simulink model "source_binaire"  (R2023b)
settings: Solver=FixedStepDiscrete  StartTime=0.0  StopTime=100000  FixedStep=1  RelTol=1e-3
values from neighbouring files (symbols this model uses):
  graine = round(P.graine)    [Parametres.m]    (also in Partie2.m = P.graine; parametres_perso.m = mod(sum(c .* (1:numel(c)) * 31) + 7 * numel(c), 2^31 - 1))
  p1 = P.p1    [Parametres.m]    (also in Partie2.m)
settings Model: Creator=e2403517  LastModifiedBy=e2403517

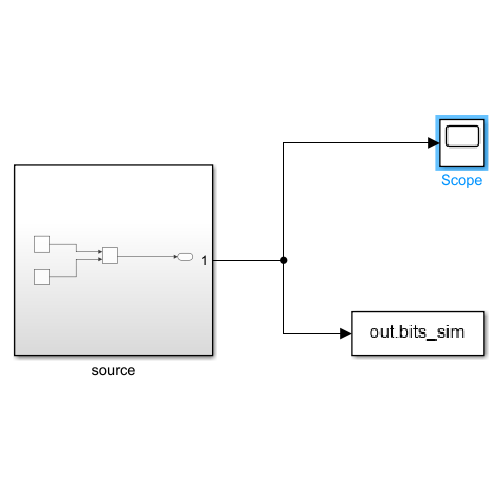
[thumbnail: Simulink's stored preview of the top-level diagram]
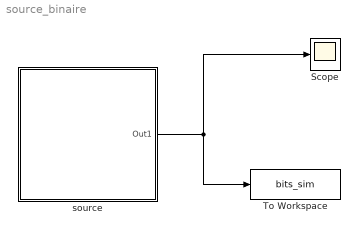
== system source_binaire ==
  Scope : Scope
  To Workspace : ToWorkspace  VariableName=bits_sim  SampleTime=1
  source : Subsystem
  wires:
  source/1(Out1) -> Scope/1, To Workspace/1

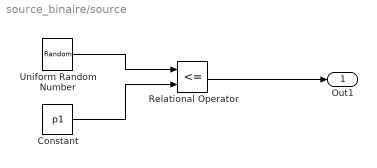
== system source_binaire/source ==
  Constant : Constant  Value=p1  SampleTime=1
  Relational Operator : RelationalOperator  Operator=<=  OutDataTypeStr=boolean  RndMeth=Simplest  InputSameDT=off
  Uniform Random Number : UniformRandomNumber  Minimum=0  Seed=graine  SampleTime=1
  Out1 : Outport
  wires:
  Uniform Random Number/1 -> Relational Operator/1
  Constant/1 -> Relational Operator/2
  Relational Operator/1 -> Out1/1
